simulink library "lib_Grid_AC_Dynamic"  (R2026a)
settings: Solver=VariableStepAuto
undefined symbols (not defined in the file): C_Lines, Cbuses, fref, From_buses, From_nodes, L_Loads, Lines_fromM, Lines_toM, Load_buses, Nbuses, op_Grid_AC_Dynamic, R_Lines, R_Loads, shift_lines, t_close_lines, tap_lines, To_buses, To_nodes
(part 2 of 2)

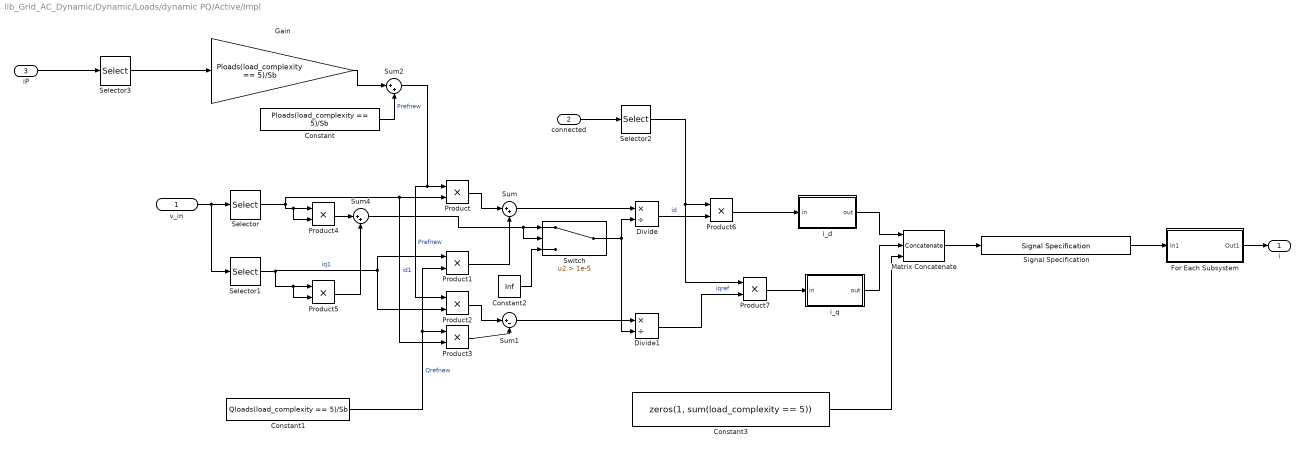
== system lib_Grid_AC_Dynamic/Dynamic/Loads/dynamic PQ/Active/Impl ==
  v_in : Inport
  connected : Inport  Port=2
  iP : Inport  Port=3
  Constant : Constant  Value=Ploads(load_complexity == 5)/Sb  VectorParams1D=off
  Constant1 : Constant  Value=Qloads(load_complexity == 5)/Sb  VectorParams1D=off
  Constant2 : Constant  Value=Inf
  Constant3 : Constant  Value=zeros(1, sum(load_complexity == 5))  VectorParams1D=off
  Divide : Product  Inputs=*/
  Divide1 : Product  Inputs=*/
  For Each Subsystem : Subsystem  TreatAsAtomicUnit=on
  Gain : Gain  Gain=Ploads(load_complexity == 5)/Sb
  Matrix Concatenate : Concatenate  NumInputs=3  Mode=Multidimensional array
  Product{,1..7} (8 alike) : Product
  Selector : Selector  NumberOfDimensions=2  InputPortWidth=3  IndexOptions=Index vector (dialog),Index vector (dialog)  Indices=1,find(load_complexity == 5)  OutputSizes=1,1
  Selector1 : Selector  NumberOfDimensions=2  InputPortWidth=3  IndexOptions=Index vector (dialog),Index vector (dialog)  Indices=2,find(load_complexity == 5)  OutputSizes=1,1
  Selector2 : Selector  InputPortWidth=length(R_Loads)  IndexOptions=Index vector (dialog)  Indices=find(load_complexity == 5)  OutputSizes=1
  Selector3 : Selector  InputPortWidth=length(R_Loads)  IndexOptions=Index vector (dialog)  Indices=find(load_complexity == 5)  OutputSizes=1
  Signal Specification : SignalSpecification  Dimensions=[3 sum(load_complexity == 5)]
  Sum : Sum  Inputs=|++
  Sum1 : Sum  Inputs=|+-
  Sum2 : Sum  Inputs=|++
  Sum4 : Sum  Inputs=|++
  Switch : Switch  Criteria=u2 > Threshold  Threshold=1e-5  ZeroCross=off  SaturateOnIntegerOverflow=off  InputSameDT=off
  i_d : Subsystem  mask{T_s=0.01}
      mask prompts: T_s "Filter time constant"
      mask Display:
      | try
      |     dpoly(1, [T_s, 1])
      | catch
      | end
  i_q : Subsystem  mask{T_s=0.01}
      mask prompts: T_s "Filter time constant"
      mask Display:
      | try
      |     dpoly(1, [T_s, 1])
      | catch
      | end
  i : Outport
  wires:
  Constant3/1 -> Matrix Concatenate/3
  Signal Specification/1 -> For Each Subsystem/1(In1)
  For Each Subsystem/1(Out1) -> i/1
  Selector3/1 -> Gain/1
  Selector2/1 -> Product6/1, Product7/1
  i_q/1(out) -> Matrix Concatenate/2
  i_d/1(out) -> Matrix Concatenate/1
  Matrix Concatenate/1 -> Signal Specification/1
  Selector1/1 -> Product5/1, Product5/2, Product2/2, Product1/1  "iq1"
  Selector/1 -> Product4/1, Product4/2, Product/2, Product3/2  "id1"
  Constant1/1 -> Product3/1, Product1/2  "Qrefnew"
  Gain/1 -> Sum2/1
  Constant/1 -> Sum2/2  "Prefnew"
  iP/1 -> Selector3/1
  Product1/1 -> Sum/2
  Product/1 -> Sum/1
  Sum2/1 -> Product/1, Product2/1  "Prefnew"
  Product2/1 -> Sum1/1
  v_in/1 -> Selector1/1, Selector/1
  Product3/1 -> Sum1/2
  Product5/1 -> Sum4/2
  Product4/1 -> Sum4/1
  Sum/1 -> Divide/1
  Switch/1 -> Divide1/2, Divide/2
  Sum4/1 -> Switch/1, Switch/2
  Constant2/1 -> Switch/3
  Sum1/1 -> Divide1/1
  connected/1 -> Selector2/1
  Divide/1 -> Product6/2  "id"
  Product6/1 -> i_d/1(in)
  Divide1/1 -> Product7/2  "iqref"
  Product7/1 -> i_q/1(in)

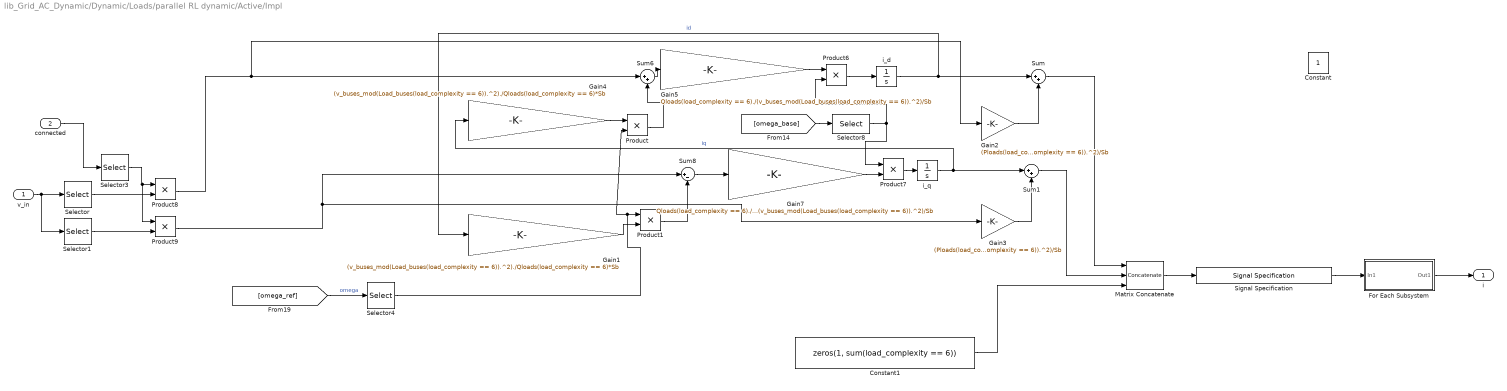
== system lib_Grid_AC_Dynamic/Dynamic/Loads/parallel RL dynamic/Active/Impl ==
  v_in : Inport
  connected : Inport  Port=2
  Constant : Constant
  Constant1 : Constant  Value=zeros(1, sum(load_complexity == 6))  VectorParams1D=off
  For Each Subsystem : Subsystem  TreatAsAtomicUnit=on
  Gain1 : Gain  Gain=(v_buses_mod(Load_buses(load_complexity == 6)).^2)./Qloads(load_complexity == 6)*Sb
  Gain2 : Gain  Gain=(Ploads(load_complexity == 6)./v_buses_mod(Load_buses(load_complexity == 6)).^2)/Sb
  Gain3 : Gain  Gain=(Ploads(load_complexity == 6)./v_buses_mod(Load_buses(load_complexity == 6)).^2)/Sb
  Gain4 : Gain  Gain=(v_buses_mod(Load_buses(load_complexity == 6)).^2)./Qloads(load_complexity == 6)*Sb
  Gain5 : Gain  Gain=Qloads(load_complexity == 6)./(v_buses_mod(Load_buses(load_complexity == 6)).^2)/Sb
  Gain7 : Gain  Gain=Qloads(load_complexity == 6)./(v_buses_mod(Load_buses(load_complexity == 6)).^2)/Sb
  Matrix Concatenate : Concatenate  NumInputs=3  Mode=Multidimensional array
  Product{,1,6..9} (6 alike) : Product
  Selector : Selector  NumberOfDimensions=2  InputPortWidth=3  IndexOptions=Index vector (dialog),Index vector (dialog)  Indices=1,find(load_complexity == 6)  OutputSizes=1,1
  Selector1 : Selector  NumberOfDimensions=2  InputPortWidth=3  IndexOptions=Index vector (dialog),Index vector (dialog)  Indices=2,find(load_complexity == 6)  OutputSizes=1,1
  Selector3 : Selector  InputPortWidth=length(R_Loads)  IndexOptions=Index vector (dialog)  Indices=find(load_complexity == 6)  OutputSizes=1
  Selector4 : Selector  InputPortWidth=length(fref.ref_units)  IndexOptions=Index vector (dialog)  Indices=fref.loads(load_complexity == 6)  OutputSizes=1
  Selector8 : Selector  InputPortWidth=length(fref.ref_units)  IndexOptions=Index vector (dialog)  Indices=fref.loads(load_complexity == 6)  OutputSizes=1
  Signal Specification : SignalSpecification  Dimensions=[3 sum(load_complexity == 6)]
  Sum : Sum  Inputs=|++
  Sum1 : Sum  Inputs=|++
  Sum6 : Sum  Inputs=|++
  Sum8 : Sum  Inputs=|+-
  i_d : Integrator  InitialCondition=op_Grid_AC_Dynamic.Loads_parallel_RL_dynamic_Active_Impl_i_d
  i_q : Integrator  InitialCondition=op_Grid_AC_Dynamic.Loads_parallel_RL_dynamic_Active_Impl_i_q
  i : Outport
  wires:
  Sum1/1 -> Matrix Concatenate/2
  Gain3/1 -> Sum1/2
  Gain2/1 -> Sum/2
  Sum/1 -> Matrix Concatenate/1
  Gain5/1 -> Product6/1
  Matrix Concatenate/1 -> Signal Specification/1
  Product8/1 -> Sum6/1, Gain2/1
  Product9/1 -> Sum8/1, Gain3/1
  Selector8/1 -> Product6/2, Product7/1
  Product/1 -> Sum6/2
  Constant1/1 -> Matrix Concatenate/3
  Product7/1 -> i_q/1
  v_in/1 -> Selector1/1, Selector/1
  Gain4/1 -> Product/1
  i_d/1 -> Gain1/1, Sum/1  "id"
  Gain7/1 -> Product7/2
  Product1/1 -> Sum8/2
  Sum6/1 -> Gain5/1
  Gain1/1 -> Product1/2
  For Each Subsystem/1(Out1) -> i/1
  [omega_base] -> Selector8/1
  connected/1 -> Selector3/1
  i_q/1 -> Gain4/1, Sum1/1  "iq"
  Selector3/1 -> Product9/1, Product8/1
  Selector1/1 -> Product9/2
  Product6/1 -> i_d/1
  Selector/1 -> Product8/2
  Signal Specification/1 -> For Each Subsystem/1(In1)
  [omega_ref] -> Selector4/1  "omega"
  Selector4/1 -> Product1/1, Product/2
  Sum8/1 -> Gain7/1

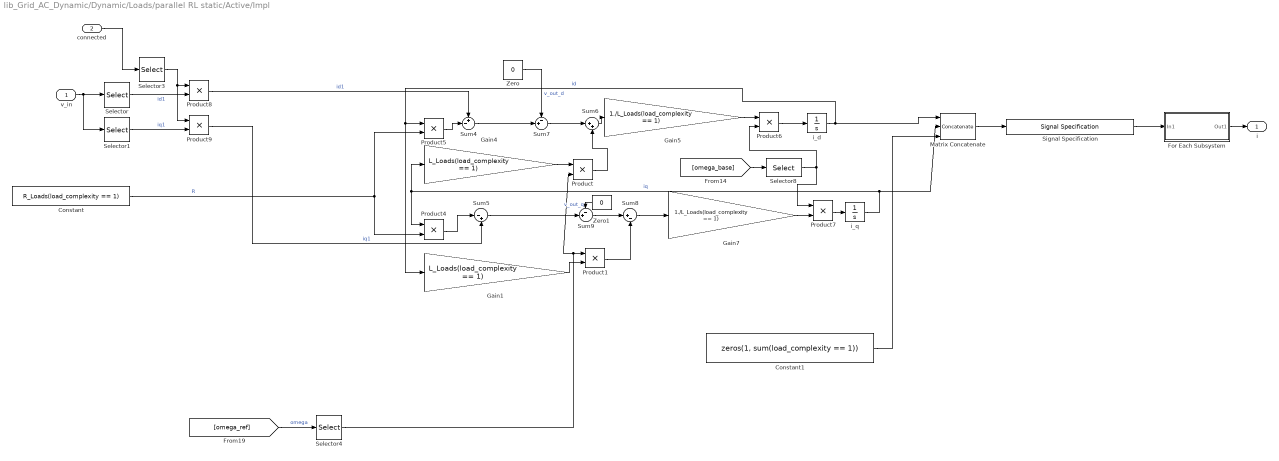
== system lib_Grid_AC_Dynamic/Dynamic/Loads/parallel RL static/Active/Impl ==
  v_in : Inport
  connected : Inport  Port=2
  Constant : Constant  Value=R_Loads(load_complexity == 1)  VectorParams1D=off
  Constant1 : Constant  Value=zeros(1, sum(load_complexity == 1))  VectorParams1D=off
  For Each Subsystem : Subsystem  TreatAsAtomicUnit=on
  Gain1 : Gain  Gain=L_Loads(load_complexity == 1)
  Gain4 : Gain  Gain=L_Loads(load_complexity == 1)
  Gain5 : Gain  Gain=1./L_Loads(load_complexity == 1)
  Gain7 : Gain  Gain=1./L_Loads(load_complexity == 1)
  Matrix Concatenate : Concatenate  NumInputs=3  Mode=Multidimensional array
  Product{,1,4..9} (8 alike) : Product
  Selector : Selector  NumberOfDimensions=2  InputPortWidth=3  IndexOptions=Index vector (dialog),Index vector (dialog)  Indices=1,find(load_complexity == 1)  OutputSizes=1,1
  Selector1 : Selector  NumberOfDimensions=2  InputPortWidth=3  IndexOptions=Index vector (dialog),Index vector (dialog)  Indices=2,find(load_complexity == 1)  OutputSizes=1,1
  Selector3 : Selector  InputPortWidth=length(R_Loads)  IndexOptions=Index vector (dialog)  Indices=find(load_complexity == 1)  OutputSizes=1
  Selector4 : Selector  InputPortWidth=length(fref.ref_units)  IndexOptions=Index vector (dialog)  Indices=fref.loads(load_complexity == 1)  OutputSizes=1
  Selector8 : Selector  InputPortWidth=length(fref.ref_units)  IndexOptions=Index vector (dialog)  Indices=fref.loads(load_complexity == 1)  OutputSizes=1
  Signal Specification : SignalSpecification  Dimensions=[3 sum(load_complexity == 1)]
  Sum4 : Sum  Inputs=+-|
  Sum5 : Sum  Inputs=|-+
  Sum6 : Sum  Inputs=|++
  Sum7 : Sum  Inputs=-+|
  Sum8 : Sum  Inputs=|+-
  Sum9 : Sum  Inputs=-+|
  Zero : Constant  Value=0  OutDataTypeStr=Inherit: Inherit via back propagation
  Zero1 : Constant  Value=0  OutDataTypeStr=Inherit: Inherit via back propagation
  i_d : Integrator  InitialCondition=op_Grid_AC_Dynamic.Loads_parallel_RL_static_Active_Impl_i_d
  i_q : Integrator  InitialCondition=op_Grid_AC_Dynamic.Loads_parallel_RL_static_Active_Impl_i_q
  i : Outport
  wires:
  Selector1/1 -> Product9/2  "iq1"
  Selector3/1 -> Product8/1, Product9/1
  Selector/1 -> Product8/2  "id1"
  connected/1 -> Selector3/1
  Product6/1 -> i_d/1
  Gain5/1 -> Product6/1
  Gain7/1 -> Product7/2
  Product7/1 -> i_q/1
  Selector8/1 -> Product7/1, Product6/2
  [omega_base] -> Selector8/1
  Selector4/1 -> Product/2, Product1/1
  Constant/1 -> Product4/2, Product5/2  "R"
  Constant1/1 -> Matrix Concatenate/3
  Signal Specification/1 -> For Each Subsystem/1(In1)
  For Each Subsystem/1(Out1) -> i/1
  Product9/1 -> Sum5/2  "iq1"
  Product8/1 -> Sum4/1  "id1"
  Matrix Concatenate/1 -> Signal Specification/1
  Zero1/1 -> Sum9/1  "v_out_q"
  Zero/1 -> Sum7/1  "v_out_d"
  Sum9/1 -> Sum8/1
  Gain1/1 -> Product1/2
  i_q/1 -> Gain4/1, Product4/1, Matrix Concatenate/2  "iq"
  Sum5/1 -> Sum9/2
  Product4/1 -> Sum5/1
  Sum7/1 -> Sum6/1
  Gain4/1 -> Product/1
  Product1/1 -> Sum8/2
  Sum4/1 -> Sum7/2
  Sum8/1 -> Gain7/1
  Product/1 -> Sum6/2
  [omega_ref] -> Selector4/1  "omega"
  Sum6/1 -> Gain5/1
  i_d/1 -> Product5/1, Gain1/1, Matrix Concatenate/1  "id"
  Product5/1 -> Sum4/2
  v_in/1 -> Selector/1, Selector1/1

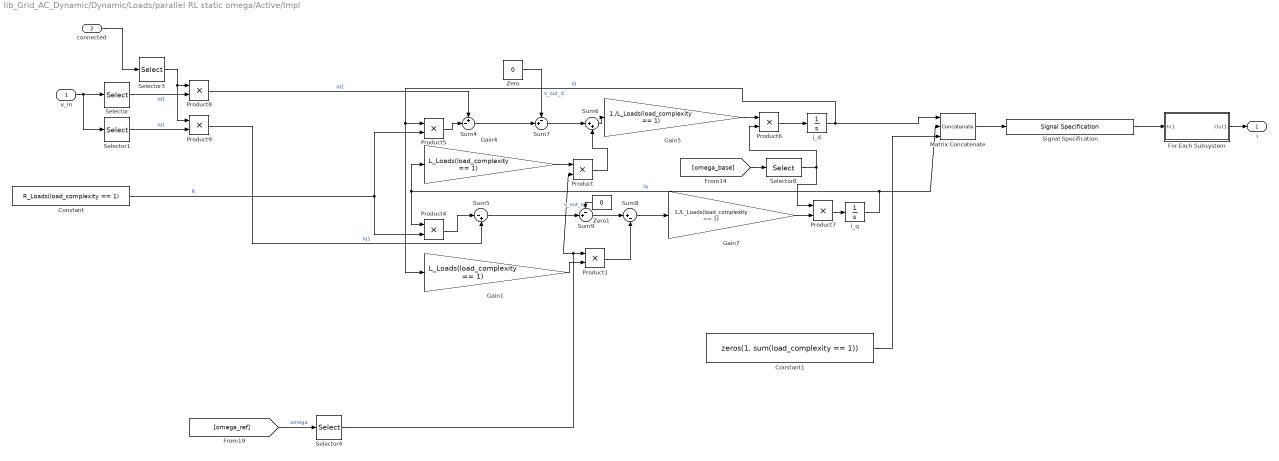
== system lib_Grid_AC_Dynamic/Dynamic/Loads/parallel RL static omega/Active/Impl ==
  v_in : Inport
  connected : Inport  Port=2
  Constant : Constant  Value=R_Loads(load_complexity == 1)  VectorParams1D=off
  Constant1 : Constant  Value=zeros(1, sum(load_complexity == 1))  VectorParams1D=off
  For Each Subsystem : Subsystem  TreatAsAtomicUnit=on
  Gain1 : Gain  Gain=L_Loads(load_complexity == 1)
  Gain4 : Gain  Gain=L_Loads(load_complexity == 1)
  Gain5 : Gain  Gain=1./L_Loads(load_complexity == 1)
  Gain7 : Gain  Gain=1./L_Loads(load_complexity == 1)
  Matrix Concatenate : Concatenate  NumInputs=3  Mode=Multidimensional array
  Product{,1,4..9} (8 alike) : Product
  Selector : Selector  NumberOfDimensions=2  InputPortWidth=3  IndexOptions=Index vector (dialog),Index vector (dialog)  Indices=1,find(load_complexity == 1)  OutputSizes=1,1
  Selector1 : Selector  NumberOfDimensions=2  InputPortWidth=3  IndexOptions=Index vector (dialog),Index vector (dialog)  Indices=2,find(load_complexity == 1)  OutputSizes=1,1
  Selector3 : Selector  InputPortWidth=length(R_Loads)  IndexOptions=Index vector (dialog)  Indices=find(load_complexity == 1)  OutputSizes=1
  Selector4 : Selector  InputPortWidth=length(fref.ref_units)  IndexOptions=Index vector (dialog)  Indices=fref.loads(load_complexity == 1)  OutputSizes=1
  Selector8 : Selector  InputPortWidth=length(fref.ref_units)  IndexOptions=Index vector (dialog)  Indices=fref.loads(load_complexity == 1)  OutputSizes=1
  Signal Specification : SignalSpecification  Dimensions=[3 sum(load_complexity == 1)]
  Sum4 : Sum  Inputs=+-|
  Sum5 : Sum  Inputs=|-+
  Sum6 : Sum  Inputs=|++
  Sum7 : Sum  Inputs=-+|
  Sum8 : Sum  Inputs=|+-
  Sum9 : Sum  Inputs=-+|
  Zero : Constant  Value=0  OutDataTypeStr=Inherit: Inherit via back propagation
  Zero1 : Constant  Value=0  OutDataTypeStr=Inherit: Inherit via back propagation
  i_d : Integrator  InitialCondition=op_Grid_AC_Dynamic.Loads_parallel_RL_static_omega_Active_Impl_i_d
  i_q : Integrator  InitialCondition=op_Grid_AC_Dynamic.Loads_parallel_RL_static_omega_Active_Impl_i_q
  i : Outport
  wires:
  v_in/1 -> Selector1/1, Selector/1
  Product5/1 -> Sum4/2
  i_d/1 -> Matrix Concatenate/1, Gain1/1, Product5/1  "id"
  Sum6/1 -> Gain5/1
  [omega_ref] -> Selector4/1  "omega"
  Product/1 -> Sum6/2
  Sum8/1 -> Gain7/1
  Sum4/1 -> Sum7/2
  Product1/1 -> Sum8/2
  Gain4/1 -> Product/1
  Sum7/1 -> Sum6/1
  Product4/1 -> Sum5/1
  Sum5/1 -> Sum9/2
  i_q/1 -> Matrix Concatenate/2, Product4/1, Gain4/1  "iq"
  Gain1/1 -> Product1/2
  Sum9/1 -> Sum8/1
  Zero/1 -> Sum7/1  "v_out_d"
  Zero1/1 -> Sum9/1  "v_out_q"
  Matrix Concatenate/1 -> Signal Specification/1
  Product8/1 -> Sum4/1  "id1"
  Product9/1 -> Sum5/2  "iq1"
  For Each Subsystem/1(Out1) -> i/1
  Signal Specification/1 -> For Each Subsystem/1(In1)
  Constant1/1 -> Matrix Concatenate/3
  Constant/1 -> Product5/2, Product4/2  "R"
  Selector4/1 -> Product1/1, Product/2
  [omega_base] -> Selector8/1
  Selector8/1 -> Product6/2, Product7/1
  Product7/1 -> i_q/1
  Gain7/1 -> Product7/2
  Gain5/1 -> Product6/1
  Product6/1 -> i_d/1
  connected/1 -> Selector3/1
  Selector/1 -> Product8/2  "id1"
  Selector3/1 -> Product9/1, Product8/1
  Selector1/1 -> Product9/2  "iq1"

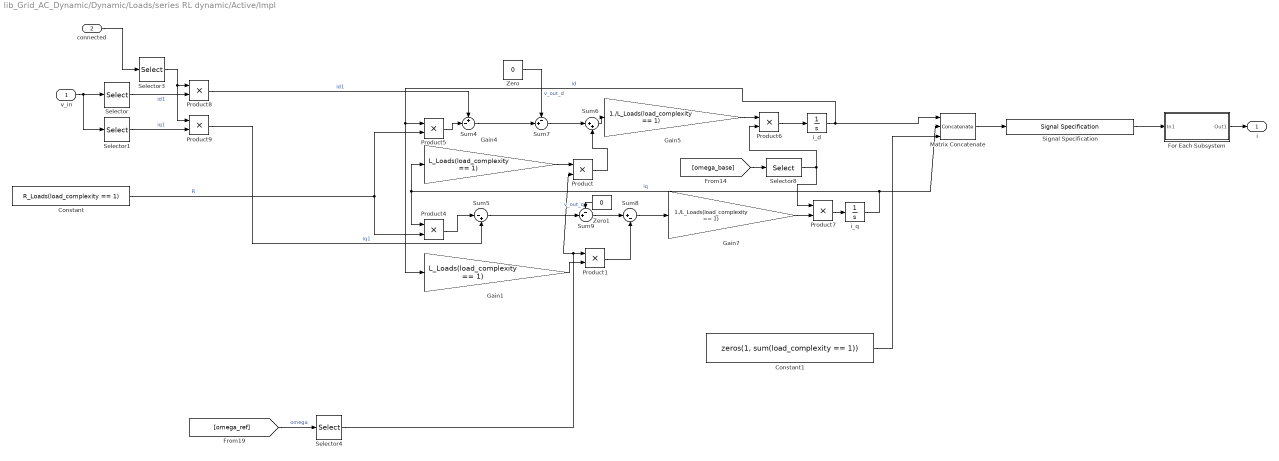
== system lib_Grid_AC_Dynamic/Dynamic/Loads/series RL dynamic/Active/Impl ==
  v_in : Inport
  connected : Inport  Port=2
  Constant : Constant  Value=R_Loads(load_complexity == 1)  VectorParams1D=off
  Constant1 : Constant  Value=zeros(1, sum(load_complexity == 1))  VectorParams1D=off
  For Each Subsystem : Subsystem  TreatAsAtomicUnit=on
  Gain1 : Gain  Gain=L_Loads(load_complexity == 1)
  Gain4 : Gain  Gain=L_Loads(load_complexity == 1)
  Gain5 : Gain  Gain=1./L_Loads(load_complexity == 1)
  Gain7 : Gain  Gain=1./L_Loads(load_complexity == 1)
  Matrix Concatenate : Concatenate  NumInputs=3  Mode=Multidimensional array
  Product{,1,4..9} (8 alike) : Product
  Selector : Selector  NumberOfDimensions=2  InputPortWidth=3  IndexOptions=Index vector (dialog),Index vector (dialog)  Indices=1,find(load_complexity == 1)  OutputSizes=1,1
  Selector1 : Selector  NumberOfDimensions=2  InputPortWidth=3  IndexOptions=Index vector (dialog),Index vector (dialog)  Indices=2,find(load_complexity == 1)  OutputSizes=1,1
  Selector3 : Selector  InputPortWidth=length(R_Loads)  IndexOptions=Index vector (dialog)  Indices=find(load_complexity == 1)  OutputSizes=1
  Selector4 : Selector  InputPortWidth=length(fref.ref_units)  IndexOptions=Index vector (dialog)  Indices=fref.loads(load_complexity == 1)  OutputSizes=1
  Selector8 : Selector  InputPortWidth=length(fref.ref_units)  IndexOptions=Index vector (dialog)  Indices=fref.loads(load_complexity == 1)  OutputSizes=1
  Signal Specification : SignalSpecification  Dimensions=[3 sum(load_complexity == 1)]
  Sum4 : Sum  Inputs=+-|
  Sum5 : Sum  Inputs=|-+
  Sum6 : Sum  Inputs=|++
  Sum7 : Sum  Inputs=-+|
  Sum8 : Sum  Inputs=|+-
  Sum9 : Sum  Inputs=-+|
  Zero : Constant  Value=0  OutDataTypeStr=Inherit: Inherit via back propagation
  Zero1 : Constant  Value=0  OutDataTypeStr=Inherit: Inherit via back propagation
  i_d : Integrator  InitialCondition=op_Grid_AC_Dynamic.Loads_series_RL_dynamic_Active_Impl_i_d
  i_q : Integrator  InitialCondition=op_Grid_AC_Dynamic.Loads_series_RL_dynamic_Active_Impl_i_q
  i : Outport
  wires:
  Product7/1 -> i_q/1
  Product6/1 -> i_d/1
  Selector1/1 -> Product9/2  "iq1"
  Selector3/1 -> Product8/1, Product9/1
  Selector/1 -> Product8/2  "id1"
  connected/1 -> Selector3/1
  Gain5/1 -> Product6/1
  Gain7/1 -> Product7/2
  Selector8/1 -> Product7/1, Product6/2
  [omega_base] -> Selector8/1
  Selector4/1 -> Product/2, Product1/1
  Constant/1 -> Product4/2, Product5/2  "R"
  Constant1/1 -> Matrix Concatenate/3
  Signal Specification/1 -> For Each Subsystem/1(In1)
  For Each Subsystem/1(Out1) -> i/1
  Product9/1 -> Sum5/2  "iq1"
  Product8/1 -> Sum4/1  "id1"
  Matrix Concatenate/1 -> Signal Specification/1
  Zero1/1 -> Sum9/1  "v_out_q"
  Zero/1 -> Sum7/1  "v_out_d"
  Sum9/1 -> Sum8/1
  Gain1/1 -> Product1/2
  i_q/1 -> Gain4/1, Product4/1, Matrix Concatenate/2  "iq"
  Sum5/1 -> Sum9/2
  Product4/1 -> Sum5/1
  Sum7/1 -> Sum6/1
  Gain4/1 -> Product/1
  Product1/1 -> Sum8/2
  Sum4/1 -> Sum7/2
  Sum8/1 -> Gain7/1
  Product/1 -> Sum6/2
  [omega_ref] -> Selector4/1  "omega"
  Sum6/1 -> Gain5/1
  i_d/1 -> Product5/1, Gain1/1, Matrix Concatenate/1  "id"
  Product5/1 -> Sum4/2
  v_in/1 -> Selector/1, Selector1/1

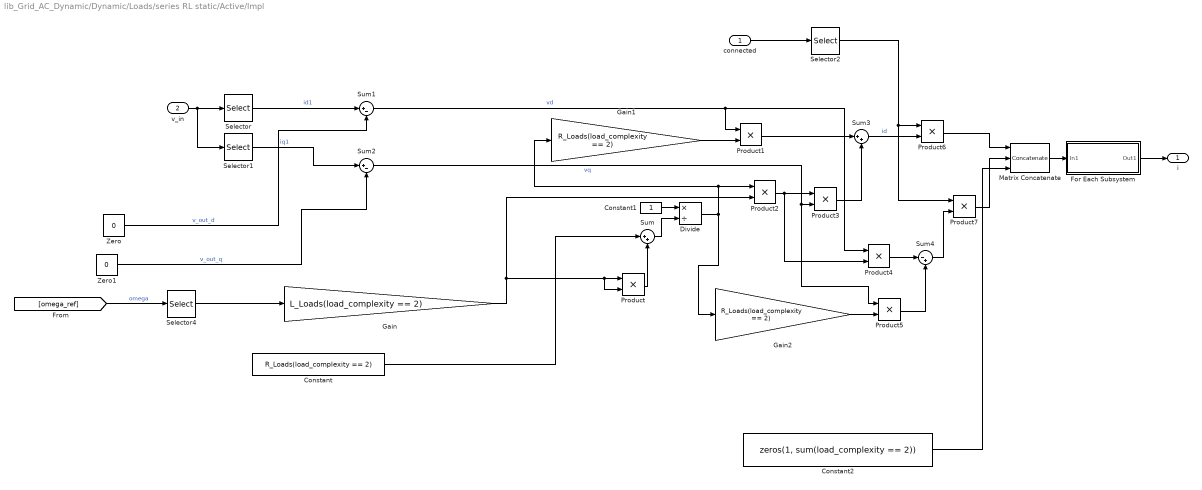
== system lib_Grid_AC_Dynamic/Dynamic/Loads/series RL static/Active/Impl ==
  connected : Inport
  v_in : Inport  Port=2
  Constant : Constant  Value=R_Loads(load_complexity == 2)  VectorParams1D=off
  Constant1 : Constant
  Constant2 : Constant  Value=zeros(1, sum(load_complexity == 2))  VectorParams1D=off
  Divide : Product  Inputs=*/
  For Each Subsystem : Subsystem  TreatAsAtomicUnit=on
  Gain : Gain  Gain=L_Loads(load_complexity == 2)
  Gain1 : Gain  Gain=R_Loads(load_complexity == 2)
  Gain2 : Gain  Gain=R_Loads(load_complexity == 2)
  Matrix Concatenate : Concatenate  NumInputs=3  Mode=Multidimensional array
  Product{,1..7} (8 alike) : Product
  Selector : Selector  NumberOfDimensions=2  InputPortWidth=3  IndexOptions=Index vector (dialog),Index vector (dialog)  Indices=1,find(load_complexity == 2)  OutputSizes=1,1
  Selector1 : Selector  NumberOfDimensions=2  InputPortWidth=3  IndexOptions=Index vector (dialog),Index vector (dialog)  Indices=2,find(load_complexity == 2)  OutputSizes=1,1
  Selector2 : Selector  InputPortWidth=length(R_Loads)  IndexOptions=Index vector (dialog)  Indices=find(load_complexity == 2)  OutputSizes=1
  Selector4 : Selector  InputPortWidth=length(fref.ref_units)  IndexOptions=Index vector (dialog)  Indices=fref.loads(load_complexity == 2)  OutputSizes=1
  Sum : Sum  Inputs=|++
  Sum1 : Sum  Inputs=|+-
  Sum2 : Sum  Inputs=|+-
  Sum3 : Sum  Inputs=|++
  Sum4 : Sum  Inputs=|-+
  Zero : Constant  Value=0  OutDataTypeStr=Inherit: Inherit via back propagation
  Zero1 : Constant  Value=0  OutDataTypeStr=Inherit: Inherit via back propagation
  i : Outport
  wires:
  Selector4/1 -> Gain/1
  Constant/1 -> Sum/1
  Constant2/1 -> Matrix Concatenate/3
  For Each Subsystem/1(Out1) -> i/1
  Selector2/1 -> Product7/1, Product6/1
  Product6/1 -> Matrix Concatenate/1
  Matrix Concatenate/1 -> For Each Subsystem/1(In1)
  Selector1/1 -> Sum2/1  "iq1"
  Selector/1 -> Sum1/1  "id1"
  Product7/1 -> Matrix Concatenate/2
  Sum4/1 -> Product7/2
  Sum3/1 -> Product6/2  "id"
  connected/1 -> Selector2/1
  [omega_ref] -> Selector4/1  "omega"
  Zero1/1 -> Sum2/2  "v_out_q"
  Gain1/1 -> Product1/2
  Product2/1 -> Product4/2, Product3/1
  Product4/1 -> Sum4/1
  Divide/1 -> Gain2/1, Gain1/1, Product2/1
  Sum1/1 -> Product1/1, Product4/1  "vd"
  Product3/1 -> Sum3/2
  Constant1/1 -> Divide/1
  Gain/1 -> Product/2, Product/1, Product2/2
  Sum2/1 -> Product5/1, Product3/2  "vq"
  Product5/1 -> Sum4/2
  Product1/1 -> Sum3/1
  Product/1 -> Sum/2
  Gain2/1 -> Product5/2
  Sum/1 -> Divide/2
  Zero/1 -> Sum1/2  "v_out_d"
  v_in/1 -> Selector/1, Selector1/1

== system lib_Grid_AC_Dynamic/Dynamic/Loads/series RL static omega/Active/Impl ==
  v_in : Inport
  connected : Inport  Port=2
  Constant1 : Constant  Value=zeros(1, sum(load_complexity == 3))  VectorParams1D=off
  For Each Subsystem : Subsystem  TreatAsAtomicUnit=on
  Gain : Gain  Gain=1./(R_Loads(load_complexity == 3).^2+L_Loads(load_complexity == 3).^2)
  Gain2 : Gain  Gain=1./(R_Loads(load_complexity == 3).^2+L_Loads(load_complexity == 3).^2)
  Gain3 : Gain  Gain=R_Loads(load_complexity == 3)
  Gain4 : Gain  Gain=L_Loads(load_complexity == 3)
  Gain5 : Gain  Gain=L_Loads(load_complexity == 3)
  Gain6 : Gain  Gain=R_Loads(load_complexity == 3)
  Matrix Concatenate : Concatenate  NumInputs=3  Mode=Multidimensional array
  Product2 : Product
  Product3 : Product
  Selector : Selector  NumberOfDimensions=2  InputPortWidth=3  IndexOptions=Index vector (dialog),Index vector (dialog)  Indices=1,find(load_complexity == 3)  OutputSizes=1,1
  Selector1 : Selector  NumberOfDimensions=2  InputPortWidth=3  IndexOptions=Index vector (dialog),Index vector (dialog)  Indices=2,find(load_complexity == 3)  OutputSizes=1,1
  Selector2 : Selector  InputPortWidth=length(R_Loads)  IndexOptions=Index vector (dialog)  Indices=find(load_complexity == 3)  OutputSizes=1
  Sum : Sum  Inputs=|++
  Sum3 : Sum  Inputs=|-+
  i : Outport
  wires:
  Constant1/1 -> Matrix Concatenate/3
  For Each Subsystem/1(Out1) -> i/1
  Selector2/1 -> Product3/1, Product2/1
  Product2/1 -> Matrix Concatenate/1
  Product3/1 -> Matrix Concatenate/2
  Matrix Concatenate/1 -> For Each Subsystem/1(In1)
  Selector1/1 -> Gain2/1  "iq1"
  Selector/1 -> Gain/1  "id1"
  Sum3/1 -> Product3/2
  Sum/1 -> Product2/2  "id"
  connected/1 -> Selector2/1
  v_in/1 -> Selector/1, Selector1/1
  Gain/1 -> Gain5/1, Gain3/1
  Gain3/1 -> Sum/1
  Gain4/1 -> Sum/2
  Gain2/1 -> Gain6/1, Gain4/1
  Gain5/1 -> Sum3/1
  Gain6/1 -> Sum3/2

== system lib_Grid_AC_Dynamic/Dynamic/Buses/dynamic/Active/Impl/For Each Subsystem ==
  In1 : Inport  Partition=on  PartitionDimension=1  PartitionWidth=1  PartitionOffset=0
  Assignment : Assignment  DiagnosticForDimensions=Warning  IndexOptions=Index vector (dialog)  Indices=find(bus_complexity == 1)  OutputSizes=1
  For Each : ForEach  DisableCoverage=on
  Zero : Constant  Value=zeros(1,Nbuses)  VectorParams1D=off  OutDataTypeStr=Inherit: Inherit via back propagation
  Out1 : Outport  ConcatenationDimension=1
  wires:
  Zero/1 -> Assignment/1
  Assignment/1 -> Out1/1
  In1/1 -> Assignment/2

== system lib_Grid_AC_Dynamic/Dynamic/Buses/only R/Active/Impl/For Each Subsystem ==
  In1 : Inport  Partition=on  PartitionDimension=1  PartitionWidth=1  PartitionOffset=0
  Assignment : Assignment  DiagnosticForDimensions=Warning  IndexOptions=Index vector (dialog)  Indices=find(bus_complexity == 4)  OutputSizes=1
  For Each : ForEach  DisableCoverage=on
  Zero : Constant  Value=zeros(1,Nbuses)  VectorParams1D=off  OutDataTypeStr=Inherit: Inherit via back propagation
  Out1 : Outport  ConcatenationDimension=1
  wires:
  Zero/1 -> Assignment/1
  Assignment/1 -> Out1/1
  In1/1 -> Assignment/2

== system lib_Grid_AC_Dynamic/Dynamic/Buses/static/Active/Impl/For Each Subsystem ==
  In1 : Inport  Partition=on  PartitionDimension=1  PartitionWidth=1  PartitionOffset=0
  Assignment : Assignment  DiagnosticForDimensions=Warning  IndexOptions=Index vector (dialog)  Indices=find(bus_complexity == 2)  OutputSizes=1
  For Each : ForEach  DisableCoverage=on
  Zero : Constant  Value=zeros(1,Nbuses)  VectorParams1D=off  OutDataTypeStr=Inherit: Inherit via back propagation
  Out1 : Outport  ConcatenationDimension=1
  wires:
  Zero/1 -> Assignment/1
  Assignment/1 -> Out1/1
  In1/1 -> Assignment/2

== system lib_Grid_AC_Dynamic/Dynamic/Buses/static omega/Active/Impl/For Each Subsystem ==
  In1 : Inport  Partition=on  PartitionDimension=1  PartitionWidth=1  PartitionOffset=0
  Assignment : Assignment  DiagnosticForDimensions=Warning  IndexOptions=Index vector (dialog)  Indices=find(bus_complexity == 3)  OutputSizes=1
  For Each : ForEach  DisableCoverage=on
  Zero : Constant  Value=zeros(1,Nbuses)  VectorParams1D=off  OutDataTypeStr=Inherit: Inherit via back propagation
  Out1 : Outport  ConcatenationDimension=1
  wires:
  Zero/1 -> Assignment/1
  Assignment/1 -> Out1/1
  In1/1 -> Assignment/2

== system lib_Grid_AC_Dynamic/Dynamic/Buses/static omega/Active/Impl/LPF ==
  in : Inport
  Gain : Gain  Gain=1e6
  I : Integrator  InitialCondition=op_Grid_AC_Dynamic.Buses_static_omega_Active_Impl_LPF_I
  Sum4 : Sum  Inputs=|+-
  out : Outport
  wires:
  I/1 -> out/1, Sum4/2
  in/1 -> Sum4/1
  Sum4/1 -> Gain/1
  Gain/1 -> I/1

== system lib_Grid_AC_Dynamic/Dynamic/Lines/dynamic/Active/Impl/For Each Subsystem ==
  In1 : Inport  Partition=on  PartitionDimension=1  PartitionWidth=1  PartitionOffset=0
  Assignment : Assignment  DiagnosticForDimensions=Warning  IndexOptions=Index vector (dialog)  Indices=find(line_complexity == 1)  OutputSizes=1
  For Each : ForEach  DisableCoverage=on
  Zero : Constant  Value=zeros(1,length(From_buses))  VectorParams1D=off  OutDataTypeStr=Inherit: Inherit via back propagation
  Out1 : Outport  ConcatenationDimension=1
  wires:
  Zero/1 -> Assignment/1
  Assignment/1 -> Out1/1
  In1/1 -> Assignment/2

== system lib_Grid_AC_Dynamic/Dynamic/Lines/static/Active/Impl/For Each Subsystem ==
  In1 : Inport  Partition=on  PartitionDimension=1  PartitionWidth=1  PartitionOffset=0
  Assignment : Assignment  DiagnosticForDimensions=Warning  IndexOptions=Index vector (dialog)  Indices=find(line_complexity == 2)  OutputSizes=1
  For Each : ForEach  DisableCoverage=on
  Zero : Constant  Value=zeros(1,length(From_buses))  VectorParams1D=off  OutDataTypeStr=Inherit: Inherit via back propagation
  Out1 : Outport  ConcatenationDimension=1
  wires:
  Zero/1 -> Assignment/1
  Assignment/1 -> Out1/1
  In1/1 -> Assignment/2

== system lib_Grid_AC_Dynamic/Dynamic/Lines/static omega/Active/Impl/For Each Subsystem ==
  In1 : Inport  Partition=on  PartitionDimension=1  PartitionWidth=1  PartitionOffset=0
  Assignment : Assignment  DiagnosticForDimensions=Warning  IndexOptions=Index vector (dialog)  Indices=find(line_complexity == 3)  OutputSizes=1
  For Each : ForEach  DisableCoverage=on
  Zero : Constant  Value=zeros(1,length(From_buses))  VectorParams1D=off  OutDataTypeStr=Inherit: Inherit via back propagation
  Out1 : Outport  ConcatenationDimension=1
  wires:
  Zero/1 -> Assignment/1
  Assignment/1 -> Out1/1
  In1/1 -> Assignment/2

== system lib_Grid_AC_Dynamic/Dynamic/Loads/PQ/Active/Impl/For Each Subsystem ==
  In1 : Inport  Partition=on  PartitionDimension=1  PartitionWidth=1  PartitionOffset=0
  Assignment : Assignment  DiagnosticForDimensions=Warning  IndexOptions=Index vector (dialog)  Indices=find(load_complexity == 4)  OutputSizes=1
  For Each : ForEach  DisableCoverage=on
  Zero : Constant  Value=zeros(1,length(L_Loads))  VectorParams1D=off  OutDataTypeStr=Inherit: Inherit via back propagation
  Out1 : Outport  ConcatenationDimension=1
  wires:
  Zero/1 -> Assignment/1
  Assignment/1 -> Out1/1
  In1/1 -> Assignment/2

== system lib_Grid_AC_Dynamic/Dynamic/Loads/dynamic PQ/Active/Impl/For Each Subsystem ==
  In1 : Inport  Partition=on  PartitionDimension=1  PartitionWidth=1  PartitionOffset=0
  Assignment : Assignment  DiagnosticForDimensions=Warning  IndexOptions=Index vector (dialog)  Indices=find(load_complexity == 5)  OutputSizes=1
  For Each : ForEach  DisableCoverage=on
  Zero : Constant  Value=zeros(1,length(L_Loads))  VectorParams1D=off  OutDataTypeStr=Inherit: Inherit via back propagation
  Out1 : Outport  ConcatenationDimension=1
  wires:
  Zero/1 -> Assignment/1
  Assignment/1 -> Out1/1
  In1/1 -> Assignment/2

== system lib_Grid_AC_Dynamic/Dynamic/Loads/dynamic PQ/Active/Impl/i_d ==
  in : Inport
  Gain : Gain  Gain=1./T_s
  I : Integrator  InitialCondition=op_Grid_AC_Dynamic.Loads_dynamic_PQ_Active_Impl_i_d_I
  Sum4 : Sum  Inputs=|+-
  out : Outport
  wires:
  I/1 -> Sum4/2, out/1
  in/1 -> Sum4/1
  Sum4/1 -> Gain/1
  Gain/1 -> I/1

== system lib_Grid_AC_Dynamic/Dynamic/Loads/dynamic PQ/Active/Impl/i_q ==
  in : Inport
  Gain : Gain  Gain=1./T_s
  I : Integrator  InitialCondition=op_Grid_AC_Dynamic.Loads_dynamic_PQ_Active_Impl_i_q_I
  Sum4 : Sum  Inputs=|+-
  out : Outport
  wires:
  Gain/1 -> I/1
  Sum4/1 -> Gain/1
  in/1 -> Sum4/1
  I/1 -> out/1, Sum4/2

== system lib_Grid_AC_Dynamic/Dynamic/Loads/parallel RL dynamic/Active/Impl/For Each Subsystem ==
  In1 : Inport  Partition=on  PartitionDimension=1  PartitionWidth=1  PartitionOffset=0
  Assignment : Assignment  DiagnosticForDimensions=Warning  IndexOptions=Index vector (dialog)  Indices=find(load_complexity == 6)  OutputSizes=1
  For Each : ForEach  DisableCoverage=on
  Zero : Constant  Value=zeros(1,length(L_Loads))  VectorParams1D=off  OutDataTypeStr=Inherit: Inherit via back propagation
  Out1 : Outport  ConcatenationDimension=1
  wires:
  In1/1 -> Assignment/2
  Assignment/1 -> Out1/1
  Zero/1 -> Assignment/1

== system lib_Grid_AC_Dynamic/Dynamic/Loads/parallel RL static/Active/Impl/For Each Subsystem ==
  In1 : Inport  Partition=on  PartitionDimension=1  PartitionWidth=1  PartitionOffset=0
  Assignment : Assignment  DiagnosticForDimensions=Warning  IndexOptions=Index vector (dialog)  Indices=find(load_complexity == 1)  OutputSizes=1
  For Each : ForEach  DisableCoverage=on
  Zero : Constant  Value=zeros(1,length(L_Loads))  VectorParams1D=off  OutDataTypeStr=Inherit: Inherit via back propagation
  Out1 : Outport  ConcatenationDimension=1
  wires:
  Zero/1 -> Assignment/1
  Assignment/1 -> Out1/1
  In1/1 -> Assignment/2

== system lib_Grid_AC_Dynamic/Dynamic/Loads/parallel RL static omega/Active/Impl/For Each Subsystem ==
  In1 : Inport  Partition=on  PartitionDimension=1  PartitionWidth=1  PartitionOffset=0
  Assignment : Assignment  DiagnosticForDimensions=Warning  IndexOptions=Index vector (dialog)  Indices=find(load_complexity == 1)  OutputSizes=1
  For Each : ForEach  DisableCoverage=on
  Zero : Constant  Value=zeros(1,length(L_Loads))  VectorParams1D=off  OutDataTypeStr=Inherit: Inherit via back propagation
  Out1 : Outport  ConcatenationDimension=1
  wires:
  In1/1 -> Assignment/2
  Assignment/1 -> Out1/1
  Zero/1 -> Assignment/1

== system lib_Grid_AC_Dynamic/Dynamic/Loads/series RL dynamic/Active/Impl/For Each Subsystem ==
  In1 : Inport  Partition=on  PartitionDimension=1  PartitionWidth=1  PartitionOffset=0
  Assignment : Assignment  DiagnosticForDimensions=Warning  IndexOptions=Index vector (dialog)  Indices=find(load_complexity == 1)  OutputSizes=1
  For Each : ForEach  DisableCoverage=on
  Zero : Constant  Value=zeros(1,length(L_Loads))  VectorParams1D=off  OutDataTypeStr=Inherit: Inherit via back propagation
  Out1 : Outport  ConcatenationDimension=1
  wires:
  Zero/1 -> Assignment/1
  Assignment/1 -> Out1/1
  In1/1 -> Assignment/2

== system lib_Grid_AC_Dynamic/Dynamic/Loads/series RL static/Active/Impl/For Each Subsystem ==
  In1 : Inport  Partition=on  PartitionDimension=1  PartitionWidth=1  PartitionOffset=0
  Assignment : Assignment  DiagnosticForDimensions=Warning  IndexOptions=Index vector (dialog)  Indices=find(load_complexity == 2)  OutputSizes=1
  For Each : ForEach  DisableCoverage=on
  Zero : Constant  Value=zeros(1,length(L_Loads))  VectorParams1D=off  OutDataTypeStr=Inherit: Inherit via back propagation
  Out1 : Outport  ConcatenationDimension=1
  wires:
  Zero/1 -> Assignment/1
  Assignment/1 -> Out1/1
  In1/1 -> Assignment/2

== system lib_Grid_AC_Dynamic/Dynamic/Loads/series RL static omega/Active/Impl/For Each Subsystem ==
  In1 : Inport  Partition=on  PartitionDimension=1  PartitionWidth=1  PartitionOffset=0
  Assignment : Assignment  DiagnosticForDimensions=Warning  IndexOptions=Index vector (dialog)  Indices=find(load_complexity == 3)  OutputSizes=1
  For Each : ForEach  DisableCoverage=on
  Zero : Constant  Value=zeros(1,length(L_Loads))  VectorParams1D=off  OutDataTypeStr=Inherit: Inherit via back propagation
  Out1 : Outport  ConcatenationDimension=1
  wires:
  Zero/1 -> Assignment/1
  Assignment/1 -> Out1/1
  In1/1 -> Assignment/2
